simulink model "si_tank_pi"  (R2025b)
settings: Solver=ode45  StartTime=0.0  StopTime=80  MaxStep=.05  RelTol=1e-3
settings Model: Creator=runner  LastModifiedBy=runner

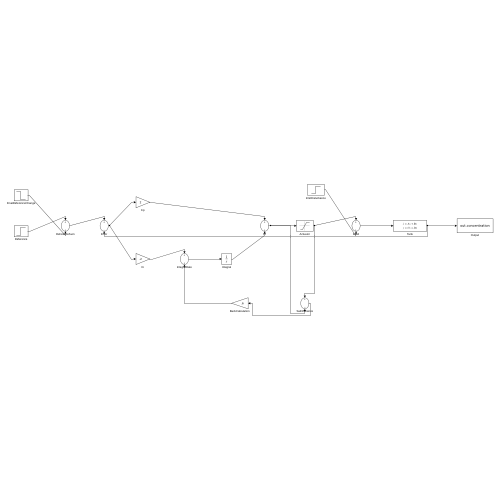
[thumbnail: Simulink's stored preview of the top-level diagram]
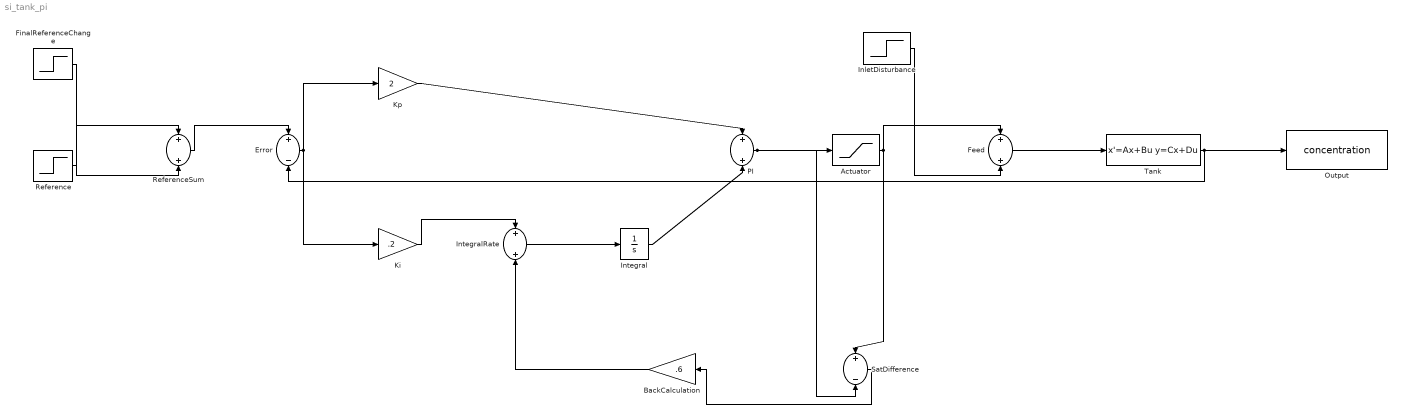
== system si_tank_pi ==
  Actuator : Saturate  UpperLimit=1  LowerLimit=0
  BackCalculation : Gain  Gain=.6
  Error : Sum  Inputs=+-
  Feed : Sum
  FinalReferenceChange : Step  Time=55  After=-.2  SampleTime=0
  InletDisturbance : Step  Time=45  After=.08  SampleTime=0
  Integral : Integrator  InitialCondition=.35
  IntegralRate : Sum
  Ki : Gain  Gain=.2
  Kp : Gain  Gain=2
  Output : ToWorkspace  VariableName=concentration  SaveFormat=Structure With Time  SampleTime=-1
  PI : Sum
  Reference : Step  Time=10  Before=.35  After=.65  SampleTime=0
  ReferenceSum : Sum
  SatDifference : Sum  Inputs=+-
  Tank : StateSpace  A=-.1  B=.1  D=0  InitialCondition=.35
  wires:
  Reference/1 -> ReferenceSum/1
  FinalReferenceChange/1 -> ReferenceSum/2
  ReferenceSum/1 -> Error/1
  Error/1 -> Kp/1, Ki/1
  Integral/1 -> PI/2
  Kp/1 -> PI/1
  PI/1 -> Actuator/1, SatDifference/2
  Actuator/1 -> Feed/1, SatDifference/1
  InletDisturbance/1 -> Feed/2
  Feed/1 -> Tank/1
  Tank/1 -> Output/1, Error/2
  Ki/1 -> IntegralRate/1
  IntegralRate/1 -> Integral/1
  SatDifference/1 -> BackCalculation/1
  BackCalculation/1 -> IntegralRate/2
